simulink model "Bossi_Emanuele_EE460S3D_R99"  (R2025a)
settings: Solver=FixedStepDiscrete  StartTime=0.0  StopTime=120  FixedStep=dt0  RelTol=1e-3  EnableMultiTasking=on
PostLoadFcn:
  | %Set the size for the model
  | set_param(gcs,'Location',[10 10 1270 970])
  | %Set the zoom factor for the model
  | set_param(gcs,'ZoomFactor','100')
InitFcn:
  | tic
  | Bossi_Emanuele_EE460_Final
  | INIT_S3D_01
StartFcn:
  | tend0=toc;
  | tic;
StopFcn:
  | tend=toc;
  | disp(['Simulation time = ' num2str(tout(end)) ' sec'])
  | disp(['Real time = ' num2str(tend) ' sec'])
  | title('DONE')
  | SCORE=round((max(0,120-tout(end)-tend0))*4+10*(40-FuelBurned)+sum(100*double(PDONE)-100*double(PDONE<.5)));
  | PlotS3D(PlotInput);
  | text(15,22,['S: ' num2str(SCORE)]);
  | % Reset color scheme back to normal defaults
  | figure()
  | blkwhitebg('w');
  | close
values from neighbouring files (symbols this model uses):
  A_obs = [ 0  1  0  0  0  0 ... (first row only)    [Bossi_Emanuele_EE460_Final.m]
  B_obs = [ 0     0     0 ... (first row only)    [Bossi_Emanuele_EE460_Final.m]
  C_obs = [ 1 0 0 0 0 0 ... (first row only)    [Bossi_Emanuele_EE460_Final.m]
  d2r = pi/180    (= 0.0174532925199)    [INIT_S3D_01.m]
  D_obs = [ 0     0     0 ... (first row only)    [Bossi_Emanuele_EE460_Final.m]
  dt = 0.01    [INIT_S3D_01.m]
  dt0 = 0.001    [INIT_S3D_01.m]
  fr = 100    [INIT_S3D_01.m]
  G = [1,  1, -1, -1,  0,  0,  0,  0 ... (first row only)    [Bossi_Emanuele_EE460_Final.m]
  G_obs = eye(6)    [Bossi_Emanuele_EE460_Final.m]
  HM_S = 250    [INIT_S3D_01.m]
  HM_U = 500    [INIT_S3D_01.m]
  J = Jbase+JC0+JF+M*(Xcg^2+Ycg^2)    [INIT_S3D_01.m]
  Jbase = JC1+4*Ja+2*Ma*da^2+2*Ma*db^2    [INIT_S3D_01.m]
  JC0 = MC0/2    (= 10.2101761242)    [INIT_S3D_01.m]
  Kdtheta = 2 * zeta_th * wn_th * J_eff    [Bossi_Emanuele_EE460_Final.m]
  Kdtheta_fail = 2 * zeta_th_fail * wn_th_fail * J_eff    [Bossi_Emanuele_EE460_Final.m]
  Kdx = 2 * zeta_xy * wn_xy * M_eff    [Bossi_Emanuele_EE460_Final.m]
  Kdx_fail = 2 * zeta_xy_fail * wn_xy_fail * M_eff    [Bossi_Emanuele_EE460_Final.m]
  Kdy = 2 * zeta_xy * wn_xy * M_eff    [Bossi_Emanuele_EE460_Final.m]
  Kdy_fail = 2 * zeta_xy_fail * wn_xy_fail * M_eff    [Bossi_Emanuele_EE460_Final.m]
  Kptheta = J_eff * wn_th^2    [Bossi_Emanuele_EE460_Final.m]
  Kptheta_fail = J_eff * wn_th_fail^2    [Bossi_Emanuele_EE460_Final.m]
  Kpx = M_eff * wn_xy^2    [Bossi_Emanuele_EE460_Final.m]
  Kpx_fail = M_eff * wn_xy_fail^2    [Bossi_Emanuele_EE460_Final.m]
  Kpy = M_eff * wn_xy^2    [Bossi_Emanuele_EE460_Final.m]
  Kpy_fail = M_eff * wn_xy_fail^2    [Bossi_Emanuele_EE460_Final.m]
  L13 = sqrt(10)    [INIT_S3D_01.m]
  L24 = sqrt(6.25)    [INIT_S3D_01.m]
  LVL = LVL12    [INIT_S3D_01.m]
  M = MC+M1+M2+M3+M4+4*Ma    [INIT_S3D_01.m]
  M1 = LVL.M1    [INIT_S3D_01.m]
  M2 = LVL.M2    [INIT_S3D_01.m]
  M3 = LVL.M3    [INIT_S3D_01.m]
  M4 = LVL.M4    [INIT_S3D_01.m]
  max_qddot = [max_qddot_x; max_qddot_y; max_qddot_theta]    [Bossi_Emanuele_EE460_Final.m]
  mdti = (1/300)    (= 0.00333333333333)    [INIT_S3D_01.m]
  P = [1  1 -1 -1  0  0  0  0 ... (first row only)    [Bossi_Emanuele_EE460_Final.m]
  Pdata = [LVL.P1 LVL.P2 LVL.P3 LVL.P4]    [INIT_S3D_01.m]    (also in PlotS3D.m = R*[xt1;yt1+[0 3*tt*TV(idx-13)*TSIG(idx-13) 0]])
  PTvec = [Pdata(:,1);Pdata(:,2);Pdata(:,3);Pdata(:,4) ... (first row only)    [INIT_S3D_01.m]
  Q_obs = eye(6)    [Bossi_Emanuele_EE460_Final.m]
  r2d = 180/pi    (= 57.2957795131)    [INIT_S3D_01.m]
  r_bang = 0.5    [Bossi_Emanuele_EE460_Final.m]
  Sconfig = 1    [Bossi_Emanuele_EE460_Final.m]
  SLIM = [-100 100 ... (first row only)    [INIT_S3D_01.m]
  SQ = [.005 .01 .004 .005 .01 .004 .02 .01 .4]'    [INIT_S3D_01.m]
  SSF = 1./SQ    [INIT_S3D_01.m]
  tau = 0.5    [Bossi_Emanuele_EE460_Final.m]
  TOLdata = [LVL.P1tol LVL.P2tol LVL.P3tol LVL.P4tol]    [INIT_S3D_01.m]
  ULIM = [[Umin Umax];0 0;0 0]    [INIT_S3D_01.m]
undefined symbols (not defined in the file or in its folder): den_lp, den_lp2, DiscIntNeverNeededParam, dt1_bang_3, dt2_bang_3, dtc_bang_3, num_lp, num_lp2, q0_1
libraries: simulink x87, matrix_library x4, sl3dlib x1, aerolibutil x1, aerolibanimutils x1
(part 5 of 8)

== system Bossi_Emanuele_EE460S3D_R99/S3D_Plant/Sensors/CASE2/Ypos1 ==
  X : Inport
  Abs : Abs  SaturateOnIntegerOverflow=off
  Bus Selector3 : BusSelector  OutputSignals=y_m
  CURRENT : Subsystem  TreatAsAtomicUnit=on
  Compare To Constant : simulink/Logic and Bit Operations/Compare To Constant  relop=<=  const=0.5  OutDataTypeStr=boolean
  Constant1 : Constant  Value=LVL.Sfail(4)  SampleTime=dt0
  Constant2 : Constant  Value=LVL.Sft(4,1)+rand*(LVL.Sft(4,2)-LVL.Sft(4,1))  SampleTime=dt0
  Digital Clock : DigitalClock  SampleTime=dt0
  Gain : Gain  Gain=LVL.SN
  If : If  IfExpression=u1 < -0.5  ElseIfExpressions=u1 > 0.5 & u1 < 1.5
  Logical Operator : Logic  Operator=OR  AllPortsSameDT=off  OutDataTypeStr=boolean
  MAX : Subsystem  TreatAsAtomicUnit=on
  MIN : Subsystem  TreatAsAtomicUnit=on
  Merge : Merge  Inputs=3
  Quantizer : Quantizer  QuantizationInterval=SQ(4)  SampleTime=dt0
  Random Number : RandomNumber  Variance=LVL.SigSense(4)  Seed=4  SampleTime=dt0
  Relational Operator : RelationalOperator  Operator=<  OutDataTypeStr=boolean  InputSameDT=off
  Saturation : Saturate  UpperLimit=SLIM(4,2)  LowerLimit=SLIM(4,1)
  Sum : Sum  Inputs=|++
  Switch : Switch  Criteria=u2 > Threshold  SaturateOnIntegerOverflow=off  InputSameDT=off
  Unit Delay : UnitDelay  SampleTime=dt0  HasFrameUpgradeWarning=on
  y1 : Outport
  wires:
  Saturation/1 -> Quantizer/1
  Compare To Constant/1 -> Logical Operator/2
  Abs/1 -> Compare To Constant/1
  Constant1/1 -> If/1, Abs/1
  Logical Operator/1 -> Switch/2
  Relational Operator/1 -> Logical Operator/1
  Sum/1 -> Switch/1
  Bus Selector3/1 -> Sum/1  "<y_m>"
  Gain/1 -> Sum/2
  Random Number/1 -> Gain/1
  Merge/1 -> Switch/3
  MIN/1(Out1) -> Merge/1
  CURRENT/1(Out1) -> Merge/3
  X/1 -> Bus Selector3/1
  Constant2/1 -> Relational Operator/2
  MAX/1(Out1) -> Merge/2
  Unit Delay/1 -> CURRENT/1(In1)
  If/3 -> CURRENT/Action
  Digital Clock/1 -> Relational Operator/1
  Switch/1 -> Saturation/1
  If/2 -> MAX/Action
  If/1 -> MIN/Action
  Quantizer/1 -> Unit Delay/1, y1/1

== system Bossi_Emanuele_EE460S3D_R99/S3D_Plant/Sensors/CASE2/Ypos2 ==
  X : Inport
  Abs : Abs  SaturateOnIntegerOverflow=off
  Bus Selector3 : BusSelector  OutputSignals=y_m
  CURRENT : Subsystem  TreatAsAtomicUnit=on
  Compare To Constant : simulink/Logic and Bit Operations/Compare To Constant  relop=<=  const=0.5  OutDataTypeStr=boolean
  Constant1 : Constant  Value=LVL.Sfail(5)  SampleTime=dt0
  Constant2 : Constant  Value=LVL.Sft(5,1)+rand*(LVL.Sft(5,2)-LVL.Sft(5,1))  SampleTime=dt0
  Digital Clock : DigitalClock  SampleTime=dt0
  Gain : Gain  Gain=LVL.SN
  If : If  IfExpression=u1 < -0.5  ElseIfExpressions=u1 > 0.5 & u1 < 1.5
  Logical Operator : Logic  Operator=OR  AllPortsSameDT=off  OutDataTypeStr=boolean
  MAX : Subsystem  TreatAsAtomicUnit=on
  MIN : Subsystem  TreatAsAtomicUnit=on
  Merge : Merge  Inputs=3
  Quantizer : Quantizer  QuantizationInterval=SQ(4)  SampleTime=dt0
  Random Number : RandomNumber  Variance=LVL.SigSense(4)  Seed=5  SampleTime=dt0
  Relational Operator : RelationalOperator  Operator=<  OutDataTypeStr=boolean  InputSameDT=off
  Saturation : Saturate  UpperLimit=SLIM(4,2)  LowerLimit=SLIM(4,1)
  Sum : Sum  Inputs=|++
  Switch : Switch  Criteria=u2 > Threshold  SaturateOnIntegerOverflow=off  InputSameDT=off
  Unit Delay : UnitDelay  SampleTime=dt0  HasFrameUpgradeWarning=on
  y1 : Outport
  wires:
  Saturation/1 -> Quantizer/1
  Quantizer/1 -> y1/1, Unit Delay/1
  If/1 -> MIN/Action
  If/2 -> MAX/Action
  Switch/1 -> Saturation/1
  Digital Clock/1 -> Relational Operator/1
  If/3 -> CURRENT/Action
  Unit Delay/1 -> CURRENT/1(In1)
  MAX/1(Out1) -> Merge/2
  Constant2/1 -> Relational Operator/2
  X/1 -> Bus Selector3/1
  CURRENT/1(Out1) -> Merge/3
  MIN/1(Out1) -> Merge/1
  Merge/1 -> Switch/3
  Random Number/1 -> Gain/1
  Gain/1 -> Sum/2
  Bus Selector3/1 -> Sum/1  "<y_m>"
  Sum/1 -> Switch/1
  Relational Operator/1 -> Logical Operator/1
  Logical Operator/1 -> Switch/2
  Constant1/1 -> Abs/1, If/1
  Abs/1 -> Compare To Constant/1
  Compare To Constant/1 -> Logical Operator/2

== system Bossi_Emanuele_EE460S3D_R99/S3D_Plant/Sensors/CASE2/Yvel ==
  X : Inport
  Abs : Abs  SaturateOnIntegerOverflow=off
  Bus Selector3 : BusSelector  OutputSignals=ydt_mps
  CURRENT : Subsystem  TreatAsAtomicUnit=on
  Compare To Constant : simulink/Logic and Bit Operations/Compare To Constant  relop=<=  const=0.5  OutDataTypeStr=boolean
  Constant1 : Constant  Value=LVL.Sfail(6)  SampleTime=dt0
  Constant2 : Constant  Value=LVL.Sft(6,1)+rand*(LVL.Sft(6,2)-LVL.Sft(6,1))  SampleTime=dt0
  Digital Clock : DigitalClock  SampleTime=dt0
  Gain : Gain  Gain=LVL.SN
  If : If  IfExpression=u1 < -0.5  ElseIfExpressions=u1 > 0.5 & u1 < 1.5
  Logical Operator : Logic  Operator=OR  AllPortsSameDT=off  OutDataTypeStr=boolean
  MAX : Subsystem  TreatAsAtomicUnit=on
  MIN : Subsystem  TreatAsAtomicUnit=on
  Merge : Merge  Inputs=3
  Quantizer : Quantizer  QuantizationInterval=SQ(5)  SampleTime=dt0
  Random Number : RandomNumber  Variance=LVL.SigSense(5)  Seed=6  SampleTime=dt0
  Relational Operator : RelationalOperator  Operator=<  OutDataTypeStr=boolean  InputSameDT=off
  Saturation : Saturate  UpperLimit=SLIM(5,2)  LowerLimit=SLIM(5,1)
  Sum : Sum  Inputs=|++
  Switch : Switch  Criteria=u2 > Threshold  SaturateOnIntegerOverflow=off  InputSameDT=off
  Unit Delay : UnitDelay  SampleTime=dt0  HasFrameUpgradeWarning=on
  ydt1 : Outport
  wires:
  Saturation/1 -> Quantizer/1
  If/1 -> MIN/Action
  If/2 -> MAX/Action
  Switch/1 -> Saturation/1
  Digital Clock/1 -> Relational Operator/1
  If/3 -> CURRENT/Action
  Unit Delay/1 -> CURRENT/1(In1)
  MAX/1(Out1) -> Merge/2
  Constant2/1 -> Relational Operator/2
  X/1 -> Bus Selector3/1
  CURRENT/1(Out1) -> Merge/3
  MIN/1(Out1) -> Merge/1
  Merge/1 -> Switch/3
  Random Number/1 -> Gain/1
  Gain/1 -> Sum/2
  Bus Selector3/1 -> Sum/1  "<ydt_mps>"
  Sum/1 -> Switch/1
  Relational Operator/1 -> Logical Operator/1
  Logical Operator/1 -> Switch/2
  Constant1/1 -> Abs/1, If/1
  Abs/1 -> Compare To Constant/1
  Compare To Constant/1 -> Logical Operator/2
  Quantizer/1 -> ydt1/1, Unit Delay/1

== system Bossi_Emanuele_EE460S3D_R99/S3D_Plant/Sensors/CASE3/THTpos1 ==
  X : Inport
  Abs : Abs  SaturateOnIntegerOverflow=off
  Bus Selector3 : BusSelector  OutputSignals=tht_rad
  CURRENT : Subsystem  TreatAsAtomicUnit=on
  Compare To Constant : simulink/Logic and Bit Operations/Compare To Constant  relop=<=  const=0.5  OutDataTypeStr=boolean
  Constant1 : Constant  Value=LVL.Sfail(7)  SampleTime=dt0
  Constant2 : Constant  Value=LVL.Sft(7,1)+rand*(LVL.Sft(7,2)-LVL.Sft(7,1))  SampleTime=dt0
  Digital Clock : DigitalClock  SampleTime=dt0
  Gain : Gain  Gain=LVL.SN
  Gain4 : Gain  Gain=r2d
  If : If  IfExpression=u1 < -0.5  ElseIfExpressions=u1 > 0.5 & u1 < 1.5
  Logical Operator : Logic  Operator=OR  AllPortsSameDT=off  OutDataTypeStr=boolean
  MAX : Subsystem  TreatAsAtomicUnit=on
  MIN : Subsystem  TreatAsAtomicUnit=on
  Merge : Merge  Inputs=3
  Quantizer : Quantizer  QuantizationInterval=SQ(7)  SampleTime=dt0
  Random Number : RandomNumber  Variance=LVL.SigSense(7)  Seed=7  SampleTime=dt0
  Relational Operator : RelationalOperator  Operator=<  OutDataTypeStr=boolean  InputSameDT=off
  Saturation : Saturate  UpperLimit=SLIM(7,2)  LowerLimit=SLIM(7,1)
  Sum : Sum  Inputs=|++
  Switch : Switch  Criteria=u2 > Threshold  SaturateOnIntegerOverflow=off  InputSameDT=off
  Unit Delay : UnitDelay  SampleTime=dt0  HasFrameUpgradeWarning=on
  tht1 : Outport
  wires:
  Saturation/1 -> Quantizer/1
  Switch/1 -> Saturation/1
  Quantizer/1 -> Unit Delay/1, tht1/1
  Gain4/1 -> Sum/1
  Compare To Constant/1 -> Logical Operator/2
  Abs/1 -> Compare To Constant/1
  Constant1/1 -> If/1, Abs/1
  Logical Operator/1 -> Switch/2
  Relational Operator/1 -> Logical Operator/1
  Sum/1 -> Switch/1
  Bus Selector3/1 -> Gain4/1  "<tht_rad>"
  Gain/1 -> Sum/2
  Random Number/1 -> Gain/1
  Merge/1 -> Switch/3
  MIN/1(Out1) -> Merge/1
  CURRENT/1(Out1) -> Merge/3
  X/1 -> Bus Selector3/1
  Constant2/1 -> Relational Operator/2
  MAX/1(Out1) -> Merge/2
  Unit Delay/1 -> CURRENT/1(In1)
  If/3 -> CURRENT/Action
  Digital Clock/1 -> Relational Operator/1
  If/2 -> MAX/Action
  If/1 -> MIN/Action

== system Bossi_Emanuele_EE460S3D_R99/S3D_Plant/Sensors/CASE3/THTpos2 ==
  X : Inport
  Abs : Abs  SaturateOnIntegerOverflow=off
  Bus Selector3 : BusSelector  OutputSignals=tht_rad
  CURRENT : Subsystem  TreatAsAtomicUnit=on
  Compare To Constant : simulink/Logic and Bit Operations/Compare To Constant  relop=<=  const=0.5  OutDataTypeStr=boolean
  Constant1 : Constant  Value=LVL.Sfail(8)  SampleTime=dt0
  Constant2 : Constant  Value=LVL.Sft(8,1)+rand*(LVL.Sft(8,2)-LVL.Sft(8,1))  SampleTime=dt0
  Digital Clock : DigitalClock  SampleTime=dt0
  Gain : Gain  Gain=LVL.SN
  Gain4 : Gain  Gain=r2d
  If : If  IfExpression=u1 < -0.5  ElseIfExpressions=u1 > 0.5 & u1 < 1.5
  Logical Operator : Logic  Operator=OR  AllPortsSameDT=off  OutDataTypeStr=boolean
  MAX : Subsystem  TreatAsAtomicUnit=on
  MIN : Subsystem  TreatAsAtomicUnit=on
  Merge : Merge  Inputs=3
  Quantizer : Quantizer  QuantizationInterval=SQ(7)  SampleTime=dt0
  Random Number : RandomNumber  Variance=LVL.SigSense(7)  Seed=8  SampleTime=dt0
  Relational Operator : RelationalOperator  Operator=<  OutDataTypeStr=boolean  InputSameDT=off
  Saturation : Saturate  UpperLimit=SLIM(7,2)  LowerLimit=SLIM(7,1)
  Sum : Sum  Inputs=|++
  Switch : Switch  Criteria=u2 > Threshold  SaturateOnIntegerOverflow=off  InputSameDT=off
  Unit Delay : UnitDelay  SampleTime=dt0  HasFrameUpgradeWarning=on
  tht1 : Outport
  wires:
  Saturation/1 -> Quantizer/1
  If/1 -> MIN/Action
  If/2 -> MAX/Action
  Digital Clock/1 -> Relational Operator/1
  If/3 -> CURRENT/Action
  Unit Delay/1 -> CURRENT/1(In1)
  MAX/1(Out1) -> Merge/2
  Constant2/1 -> Relational Operator/2
  X/1 -> Bus Selector3/1
  CURRENT/1(Out1) -> Merge/3
  MIN/1(Out1) -> Merge/1
  Merge/1 -> Switch/3
  Random Number/1 -> Gain/1
  Gain/1 -> Sum/2
  Bus Selector3/1 -> Gain4/1  "<tht_rad>"
  Sum/1 -> Switch/1
  Relational Operator/1 -> Logical Operator/1
  Logical Operator/1 -> Switch/2
  Constant1/1 -> Abs/1, If/1
  Abs/1 -> Compare To Constant/1
  Compare To Constant/1 -> Logical Operator/2
  Gain4/1 -> Sum/1
  Switch/1 -> Saturation/1
  Quantizer/1 -> Unit Delay/1, tht1/1

== system Bossi_Emanuele_EE460S3D_R99/S3D_Plant/Sensors/CASE3/THTpos3 ==
  X : Inport
  Abs : Abs  SaturateOnIntegerOverflow=off
  Bus Selector3 : BusSelector  OutputSignals=tht_rad
  CURRENT : Subsystem  TreatAsAtomicUnit=on
  Compare To Constant : simulink/Logic and Bit Operations/Compare To Constant  relop=<=  const=0.5  OutDataTypeStr=boolean
  Constant1 : Constant  Value=LVL.Sfail(9)  SampleTime=dt0
  Constant2 : Constant  Value=LVL.Sft(9,1)+rand*(LVL.Sft(9,2)-LVL.Sft(9,1))  SampleTime=dt0
  Digital Clock : DigitalClock  SampleTime=dt0
  Gain : Gain  Gain=LVL.SN
  Gain4 : Gain  Gain=r2d
  If : If  IfExpression=u1 < -0.5  ElseIfExpressions=u1 > 0.5 & u1 < 1.5
  Logical Operator : Logic  Operator=OR  AllPortsSameDT=off  OutDataTypeStr=boolean
  MAX : Subsystem  TreatAsAtomicUnit=on
  MIN : Subsystem  TreatAsAtomicUnit=on
  Merge : Merge  Inputs=3
  Quantizer : Quantizer  QuantizationInterval=SQ(7)  SampleTime=dt0
  Random Number : RandomNumber  Variance=LVL.SigSense(7)  Seed=9  SampleTime=dt0
  Relational Operator : RelationalOperator  Operator=<  OutDataTypeStr=boolean  InputSameDT=off
  Saturation : Saturate  UpperLimit=SLIM(7,2)  LowerLimit=SLIM(7,1)
  Sum : Sum  Inputs=|++
  Switch : Switch  Criteria=u2 > Threshold  SaturateOnIntegerOverflow=off  InputSameDT=off
  Unit Delay : UnitDelay  SampleTime=dt0  HasFrameUpgradeWarning=on
  tht1 : Outport
  wires:
  Saturation/1 -> Quantizer/1
  Switch/1 -> Saturation/1
  Quantizer/1 -> Unit Delay/1, tht1/1
  Gain4/1 -> Sum/1
  Compare To Constant/1 -> Logical Operator/2
  Abs/1 -> Compare To Constant/1
  Constant1/1 -> If/1, Abs/1
  Logical Operator/1 -> Switch/2
  Relational Operator/1 -> Logical Operator/1
  Sum/1 -> Switch/1
  Bus Selector3/1 -> Gain4/1  "<tht_rad>"
  Gain/1 -> Sum/2
  Random Number/1 -> Gain/1
  Merge/1 -> Switch/3
  MIN/1(Out1) -> Merge/1
  CURRENT/1(Out1) -> Merge/3
  X/1 -> Bus Selector3/1
  Constant2/1 -> Relational Operator/2
  MAX/1(Out1) -> Merge/2
  Unit Delay/1 -> CURRENT/1(In1)
  If/3 -> CURRENT/Action
  Digital Clock/1 -> Relational Operator/1
  If/2 -> MAX/Action
  If/1 -> MIN/Action

== system Bossi_Emanuele_EE460S3D_R99/S3D_Plant/Sensors/CASE3/Xpos1 ==
  X : Inport
  Abs : Abs  SaturateOnIntegerOverflow=off
  Bus Selector3 : BusSelector  OutputSignals=x_m
  CURRENT : Subsystem  TreatAsAtomicUnit=on
  Compare To Constant : simulink/Logic and Bit Operations/Compare To Constant  relop=<=  const=0.5  OutDataTypeStr=boolean
  Constant1 : Constant  Value=LVL.Sfail(1)  SampleTime=dt0
  Constant2 : Constant  Value=LVL.Sft(1,1)+rand*(LVL.Sft(1,2)-LVL.Sft(1,1))  SampleTime=dt0
  Digital Clock : DigitalClock  SampleTime=dt0
  Gain : Gain  Gain=LVL.SN
  If : If  IfExpression=u1 < -0.5  ElseIfExpressions=u1 > 0.5 & u1 < 1.5
  Logical Operator : Logic  Operator=OR  AllPortsSameDT=off  OutDataTypeStr=boolean
  MAX : Subsystem  TreatAsAtomicUnit=on
  MIN : Subsystem  TreatAsAtomicUnit=on
  Merge : Merge  Inputs=3
  Quantizer : Quantizer  QuantizationInterval=SQ(1)  SampleTime=dt0
  Random Number : RandomNumber  Variance=LVL.SigSense(1)  Seed=1  SampleTime=dt0
  Relational Operator : RelationalOperator  Operator=<  OutDataTypeStr=boolean  InputSameDT=off
  Saturation : Saturate  UpperLimit=SLIM(1,2)  LowerLimit=SLIM(1,1)
  Sum : Sum  Inputs=|++
  Switch : Switch  Criteria=u2 > Threshold  SaturateOnIntegerOverflow=off  InputSameDT=off
  Unit Delay : UnitDelay  SampleTime=dt0  HasFrameUpgradeWarning=on
  x1 : Outport
  wires:
  Saturation/1 -> Quantizer/1
  Quantizer/1 -> Unit Delay/1, x1/1
  Compare To Constant/1 -> Logical Operator/2
  Abs/1 -> Compare To Constant/1
  Constant1/1 -> If/1, Abs/1
  Logical Operator/1 -> Switch/2
  Relational Operator/1 -> Logical Operator/1
  Sum/1 -> Switch/1
  Bus Selector3/1 -> Sum/1  "<x_m>"
  Gain/1 -> Sum/2
  Random Number/1 -> Gain/1
  Merge/1 -> Switch/3
  MIN/1(Out1) -> Merge/1
  CURRENT/1(Out1) -> Merge/3
  X/1 -> Bus Selector3/1
  Constant2/1 -> Relational Operator/2
  MAX/1(Out1) -> Merge/2
  Unit Delay/1 -> CURRENT/1(In1)
  If/3 -> CURRENT/Action
  Digital Clock/1 -> Relational Operator/1
  Switch/1 -> Saturation/1
  If/2 -> MAX/Action
  If/1 -> MIN/Action

== system Bossi_Emanuele_EE460S3D_R99/S3D_Plant/Sensors/CASE3/Xpos2 ==
  X : Inport
  Abs : Abs  SaturateOnIntegerOverflow=off
  Bus Selector3 : BusSelector  OutputSignals=x_m
  CURRENT : Subsystem  TreatAsAtomicUnit=on
  Compare To Constant : simulink/Logic and Bit Operations/Compare To Constant  relop=<=  const=0.5  OutDataTypeStr=boolean
  Constant1 : Constant  Value=LVL.Sfail(2)  SampleTime=dt0
  Constant2 : Constant  Value=LVL.Sft(2,1)+rand*(LVL.Sft(2,2)-LVL.Sft(2,1))  SampleTime=dt0
  Digital Clock : DigitalClock  SampleTime=dt0
  Gain : Gain  Gain=LVL.SN
  If : If  IfExpression=u1 < -0.5  ElseIfExpressions=u1 > 0.5 & u1 < 1.5
  Logical Operator : Logic  Operator=OR  AllPortsSameDT=off  OutDataTypeStr=boolean
  MAX : Subsystem  TreatAsAtomicUnit=on
  MIN : Subsystem  TreatAsAtomicUnit=on
  Merge : Merge  Inputs=3
  Quantizer : Quantizer  QuantizationInterval=SQ(1)  SampleTime=dt0
  Random Number : RandomNumber  Variance=LVL.SigSense(1)  Seed=2  SampleTime=dt0
  Relational Operator : RelationalOperator  Operator=<  OutDataTypeStr=boolean  InputSameDT=off
  Saturation : Saturate  UpperLimit=SLIM(1,2)  LowerLimit=SLIM(1,1)
  Sum : Sum  Inputs=|++
  Switch : Switch  Criteria=u2 > Threshold  SaturateOnIntegerOverflow=off  InputSameDT=off
  Unit Delay : UnitDelay  SampleTime=dt0  HasFrameUpgradeWarning=on
  xdt1 : Outport
  wires:
  Saturation/1 -> Quantizer/1
  Quantizer/1 -> xdt1/1, Unit Delay/1
  If/1 -> MIN/Action
  If/2 -> MAX/Action
  Switch/1 -> Saturation/1
  Digital Clock/1 -> Relational Operator/1
  If/3 -> CURRENT/Action
  Unit Delay/1 -> CURRENT/1(In1)
  MAX/1(Out1) -> Merge/2
  Constant2/1 -> Relational Operator/2
  X/1 -> Bus Selector3/1
  CURRENT/1(Out1) -> Merge/3
  MIN/1(Out1) -> Merge/1
  Merge/1 -> Switch/3
  Random Number/1 -> Gain/1
  Gain/1 -> Sum/2
  Bus Selector3/1 -> Sum/1  "<x_m>"
  Sum/1 -> Switch/1
  Relational Operator/1 -> Logical Operator/1
  Logical Operator/1 -> Switch/2
  Constant1/1 -> Abs/1, If/1
  Abs/1 -> Compare To Constant/1
  Compare To Constant/1 -> Logical Operator/2

== system Bossi_Emanuele_EE460S3D_R99/S3D_Plant/Sensors/CASE3/Xpos3 ==
  X : Inport
  Abs : Abs  SaturateOnIntegerOverflow=off
  Bus Selector3 : BusSelector  OutputSignals=x_m
  CURRENT : Subsystem  TreatAsAtomicUnit=on
  Compare To Constant : simulink/Logic and Bit Operations/Compare To Constant  relop=<=  const=0.5  OutDataTypeStr=boolean
  Constant1 : Constant  Value=LVL.Sfail(3)  SampleTime=dt0
  Constant2 : Constant  Value=LVL.Sft(3,1)+rand*(LVL.Sft(3,2)-LVL.Sft(3,1))  SampleTime=dt0
  Digital Clock : DigitalClock  SampleTime=dt0
  Gain : Gain  Gain=LVL.SN
  If : If  IfExpression=u1 < -0.5  ElseIfExpressions=u1 > 0.5 & u1 < 1.5
  Logical Operator : Logic  Operator=OR  AllPortsSameDT=off  OutDataTypeStr=boolean
  MAX : Subsystem  TreatAsAtomicUnit=on
  MIN : Subsystem  TreatAsAtomicUnit=on
  Merge : Merge  Inputs=3
  Quantizer : Quantizer  QuantizationInterval=SQ(1)  SampleTime=dt0
  Random Number : RandomNumber  Variance=LVL.SigSense(1)  Seed=3  SampleTime=dt0
  Relational Operator : RelationalOperator  Operator=<  OutDataTypeStr=boolean  InputSameDT=off
  Saturation : Saturate  UpperLimit=SLIM(1,2)  LowerLimit=SLIM(1,1)
  Sum : Sum  Inputs=|++
  Switch : Switch  Criteria=u2 > Threshold  SaturateOnIntegerOverflow=off  InputSameDT=off
  Unit Delay : UnitDelay  SampleTime=dt0  HasFrameUpgradeWarning=on
  xddt1 : Outport
  wires:
  Saturation/1 -> Quantizer/1
  Quantizer/1 -> Unit Delay/1, xddt1/1
  Compare To Constant/1 -> Logical Operator/2
  Abs/1 -> Compare To Constant/1
  Constant1/1 -> If/1, Abs/1
  Logical Operator/1 -> Switch/2
  Relational Operator/1 -> Logical Operator/1
  Sum/1 -> Switch/1
  Bus Selector3/1 -> Sum/1  "<x_m>"
  Gain/1 -> Sum/2
  Random Number/1 -> Gain/1
  Merge/1 -> Switch/3
  MIN/1(Out1) -> Merge/1
  CURRENT/1(Out1) -> Merge/3
  X/1 -> Bus Selector3/1
  Constant2/1 -> Relational Operator/2
  MAX/1(Out1) -> Merge/2
  Unit Delay/1 -> CURRENT/1(In1)
  If/3 -> CURRENT/Action
  Digital Clock/1 -> Relational Operator/1
  Switch/1 -> Saturation/1
  If/2 -> MAX/Action
  If/1 -> MIN/Action

== system Bossi_Emanuele_EE460S3D_R99/S3D_Plant/Sensors/CASE3/Ypos1 ==
  X : Inport
  Abs : Abs  SaturateOnIntegerOverflow=off
  Bus Selector3 : BusSelector  OutputSignals=y_m
  CURRENT : Subsystem  TreatAsAtomicUnit=on
  Compare To Constant : simulink/Logic and Bit Operations/Compare To Constant  relop=<=  const=0.5  OutDataTypeStr=boolean
  Constant1 : Constant  Value=LVL.Sfail(4)  SampleTime=dt0
  Constant2 : Constant  Value=LVL.Sft(4,1)+rand*(LVL.Sft(4,2)-LVL.Sft(4,1))  SampleTime=dt0
  Digital Clock : DigitalClock  SampleTime=dt0
  Gain : Gain  Gain=LVL.SN
  If : If  IfExpression=u1 < -0.5  ElseIfExpressions=u1 > 0.5 & u1 < 1.5
  Logical Operator : Logic  Operator=OR  AllPortsSameDT=off  OutDataTypeStr=boolean
  MAX : Subsystem  TreatAsAtomicUnit=on
  MIN : Subsystem  TreatAsAtomicUnit=on
  Merge : Merge  Inputs=3
  Quantizer : Quantizer  QuantizationInterval=SQ(4)  SampleTime=dt0
  Random Number : RandomNumber  Variance=LVL.SigSense(4)  Seed=4  SampleTime=dt0
  Relational Operator : RelationalOperator  Operator=<  OutDataTypeStr=boolean  InputSameDT=off
  Saturation : Saturate  UpperLimit=SLIM(4,2)  LowerLimit=SLIM(4,1)
  Sum : Sum  Inputs=|++
  Switch : Switch  Criteria=u2 > Threshold  SaturateOnIntegerOverflow=off  InputSameDT=off
  Unit Delay : UnitDelay  SampleTime=dt0  HasFrameUpgradeWarning=on
  y1 : Outport
  wires:
  Saturation/1 -> Quantizer/1
  Quantizer/1 -> y1/1, Unit Delay/1
  If/1 -> MIN/Action
  If/2 -> MAX/Action
  Switch/1 -> Saturation/1
  Digital Clock/1 -> Relational Operator/1
  If/3 -> CURRENT/Action
  Unit Delay/1 -> CURRENT/1(In1)
  MAX/1(Out1) -> Merge/2
  Constant2/1 -> Relational Operator/2
  X/1 -> Bus Selector3/1
  CURRENT/1(Out1) -> Merge/3
  MIN/1(Out1) -> Merge/1
  Merge/1 -> Switch/3
  Random Number/1 -> Gain/1
  Gain/1 -> Sum/2
  Bus Selector3/1 -> Sum/1  "<y_m>"
  Sum/1 -> Switch/1
  Relational Operator/1 -> Logical Operator/1
  Logical Operator/1 -> Switch/2
  Constant1/1 -> Abs/1, If/1
  Abs/1 -> Compare To Constant/1
  Compare To Constant/1 -> Logical Operator/2

== system Bossi_Emanuele_EE460S3D_R99/S3D_Plant/Sensors/CASE3/Ypos2 ==
  X : Inport
  Abs : Abs  SaturateOnIntegerOverflow=off
  Bus Selector3 : BusSelector  OutputSignals=y_m
  CURRENT : Subsystem  TreatAsAtomicUnit=on
  Compare To Constant : simulink/Logic and Bit Operations/Compare To Constant  relop=<=  const=0.5  OutDataTypeStr=boolean
  Constant1 : Constant  Value=LVL.Sfail(5)  SampleTime=dt0
  Constant2 : Constant  Value=LVL.Sft(5,1)+rand*(LVL.Sft(5,2)-LVL.Sft(5,1))  SampleTime=dt0
  Digital Clock : DigitalClock  SampleTime=dt0
  Gain : Gain  Gain=LVL.SN
  If : If  IfExpression=u1 < -0.5  ElseIfExpressions=u1 > 0.5 & u1 < 1.5
  Logical Operator : Logic  Operator=OR  AllPortsSameDT=off  OutDataTypeStr=boolean
  MAX : Subsystem  TreatAsAtomicUnit=on
  MIN : Subsystem  TreatAsAtomicUnit=on
  Merge : Merge  Inputs=3
  Quantizer : Quantizer  QuantizationInterval=SQ(4)  SampleTime=dt0
  Random Number : RandomNumber  Variance=LVL.SigSense(4)  Seed=5  SampleTime=dt0
  Relational Operator : RelationalOperator  Operator=<  OutDataTypeStr=boolean  InputSameDT=off
  Saturation : Saturate  UpperLimit=SLIM(4,2)  LowerLimit=SLIM(4,1)
  Sum : Sum  Inputs=|++
  Switch : Switch  Criteria=u2 > Threshold  SaturateOnIntegerOverflow=off  InputSameDT=off
  Unit Delay : UnitDelay  SampleTime=dt0  HasFrameUpgradeWarning=on
  y1 : Outport
  wires:
  Saturation/1 -> Quantizer/1
  Compare To Constant/1 -> Logical Operator/2
  Abs/1 -> Compare To Constant/1
  Constant1/1 -> If/1, Abs/1
  Logical Operator/1 -> Switch/2
  Relational Operator/1 -> Logical Operator/1
  Sum/1 -> Switch/1
  Bus Selector3/1 -> Sum/1  "<y_m>"
  Gain/1 -> Sum/2
  Random Number/1 -> Gain/1
  Merge/1 -> Switch/3
  MIN/1(Out1) -> Merge/1
  CURRENT/1(Out1) -> Merge/3
  X/1 -> Bus Selector3/1
  Constant2/1 -> Relational Operator/2
  MAX/1(Out1) -> Merge/2
  Unit Delay/1 -> CURRENT/1(In1)
  If/3 -> CURRENT/Action
  Digital Clock/1 -> Relational Operator/1
  Switch/1 -> Saturation/1
  If/2 -> MAX/Action
  If/1 -> MIN/Action
  Quantizer/1 -> Unit Delay/1, y1/1

== system Bossi_Emanuele_EE460S3D_R99/S3D_Plant/Sensors/CASE3/Ypos3 ==
  X : Inport
  Abs : Abs  SaturateOnIntegerOverflow=off
  Bus Selector3 : BusSelector  OutputSignals=y_m
  CURRENT : Subsystem  TreatAsAtomicUnit=on
  Compare To Constant : simulink/Logic and Bit Operations/Compare To Constant  relop=<=  const=0.5  OutDataTypeStr=boolean
  Constant1 : Constant  Value=LVL.Sfail(6)  SampleTime=dt0
  Constant2 : Constant  Value=LVL.Sft(6,1)+rand*(LVL.Sft(6,2)-LVL.Sft(6,1))  SampleTime=dt0
  Digital Clock : DigitalClock  SampleTime=dt0
  Gain : Gain  Gain=LVL.SN
  If : If  IfExpression=u1 < -0.5  ElseIfExpressions=u1 > 0.5 & u1 < 1.5
  Logical Operator : Logic  Operator=OR  AllPortsSameDT=off  OutDataTypeStr=boolean
  MAX : Subsystem  TreatAsAtomicUnit=on
  MIN : Subsystem  TreatAsAtomicUnit=on
  Merge : Merge  Inputs=3
  Quantizer : Quantizer  QuantizationInterval=SQ(4)  SampleTime=dt0
  Random Number : RandomNumber  Variance=LVL.SigSense(4)  Seed=6  SampleTime=dt0
  Relational Operator : RelationalOperator  Operator=<  OutDataTypeStr=boolean  InputSameDT=off
  Saturation : Saturate  UpperLimit=SLIM(4,2)  LowerLimit=SLIM(4,1)
  Sum : Sum  Inputs=|++
  Switch : Switch  Criteria=u2 > Threshold  SaturateOnIntegerOverflow=off  InputSameDT=off
  Unit Delay : UnitDelay  SampleTime=dt0  HasFrameUpgradeWarning=on
  y1 : Outport
  wires:
  Saturation/1 -> Quantizer/1
  Quantizer/1 -> y1/1, Unit Delay/1
  If/1 -> MIN/Action
  If/2 -> MAX/Action
  Switch/1 -> Saturation/1
  Digital Clock/1 -> Relational Operator/1
  If/3 -> CURRENT/Action
  Unit Delay/1 -> CURRENT/1(In1)
  MAX/1(Out1) -> Merge/2
  Constant2/1 -> Relational Operator/2
  X/1 -> Bus Selector3/1
  CURRENT/1(Out1) -> Merge/3
  MIN/1(Out1) -> Merge/1
  Merge/1 -> Switch/3
  Random Number/1 -> Gain/1
  Gain/1 -> Sum/2
  Bus Selector3/1 -> Sum/1  "<y_m>"
  Sum/1 -> Switch/1
  Relational Operator/1 -> Logical Operator/1
  Logical Operator/1 -> Switch/2
  Constant1/1 -> Abs/1, If/1
  Abs/1 -> Compare To Constant/1
  Compare To Constant/1 -> Logical Operator/2

== system Bossi_Emanuele_EE460S3D_R99/S3D_Plant/Sensors/HealthMonitoring/Subsystem ==
  In1 : Inport
  Compare To Constant : simulink/Logic and Bit Operations/Compare To Constant  relop=>=  const=HM_S  OutDataTypeStr=boolean
  Constant : Constant  Value=0
  Constant1 : Constant
  Logical Operator : Logic  Operator=OR  AllPortsSameDT=off  OutDataTypeStr=boolean
  Sum : Sum  Inputs=|+-  OutDataTypeStr=int32
  Sum1 : Sum  Inputs=|++
  Switch : Switch  Criteria=u2 > Threshold  Threshold=eps  SaturateOnIntegerOverflow=off  InputSameDT=off
  Unit Delay : UnitDelay  SampleTime=dt0  HasFrameUpgradeWarning=on
  Unit Delay1 : UnitDelay  SampleTime=dt0  HasFrameUpgradeWarning=on
  Unit Delay2 : UnitDelay  SampleTime=dt0  HasFrameUpgradeWarning=on
  Out1 : Outport
  wires:
  Logical Operator/1 -> Unit Delay2/1, Out1/1
  Constant1/1 -> Sum1/1
  Compare To Constant/1 -> Logical Operator/1
  Switch/1 -> Unit Delay1/1, Compare To Constant/1
  In1/1 -> Sum/1, Unit Delay/1
  Unit Delay2/1 -> Logical Operator/2
  Unit Delay/1 -> Sum/2
  Sum/1 -> Switch/2
  Sum1/1 -> Switch/3
  Unit Delay1/1 -> Sum1/2
  Constant/1 -> Switch/1

== system Bossi_Emanuele_EE460S3D_R99/S3D_Plant/Sensors/HealthMonitoring/Subsystem1 ==
  In1 : Inport
  Compare To Constant : simulink/Logic and Bit Operations/Compare To Constant  relop=>=  const=HM_S  OutDataTypeStr=boolean
  Constant : Constant  Value=0
  Constant1 : Constant
  Logical Operator : Logic  Operator=OR  AllPortsSameDT=off  OutDataTypeStr=boolean
  Sum : Sum  Inputs=|+-  OutDataTypeStr=int32
  Sum1 : Sum  Inputs=|++
  Switch : Switch  Criteria=u2 > Threshold  Threshold=eps  SaturateOnIntegerOverflow=off  InputSameDT=off
  Unit Delay : UnitDelay  SampleTime=dt0  HasFrameUpgradeWarning=on
  Unit Delay1 : UnitDelay  SampleTime=dt0  HasFrameUpgradeWarning=on
  Unit Delay2 : UnitDelay  SampleTime=dt0  HasFrameUpgradeWarning=on
  Out1 : Outport
  wires:
  Constant/1 -> Switch/1
  Unit Delay1/1 -> Sum1/2
  Sum1/1 -> Switch/3
  Sum/1 -> Switch/2
  Unit Delay/1 -> Sum/2
  Unit Delay2/1 -> Logical Operator/2
  In1/1 -> Unit Delay/1, Sum/1
  Switch/1 -> Compare To Constant/1, Unit Delay1/1
  Compare To Constant/1 -> Logical Operator/1
  Constant1/1 -> Sum1/1
  Logical Operator/1 -> Out1/1, Unit Delay2/1

== system Bossi_Emanuele_EE460S3D_R99/S3D_Plant/Sensors/HealthMonitoring/Subsystem2 ==
  In1 : Inport
  Compare To Constant : simulink/Logic and Bit Operations/Compare To Constant  relop=>=  const=HM_S  OutDataTypeStr=boolean
  Constant : Constant  Value=0
  Constant1 : Constant
  Logical Operator : Logic  Operator=OR  AllPortsSameDT=off  OutDataTypeStr=boolean
  Sum : Sum  Inputs=|+-  OutDataTypeStr=int32
  Sum1 : Sum  Inputs=|++
  Switch : Switch  Criteria=u2 > Threshold  Threshold=eps  SaturateOnIntegerOverflow=off  InputSameDT=off
  Unit Delay : UnitDelay  SampleTime=dt0  HasFrameUpgradeWarning=on
  Unit Delay1 : UnitDelay  SampleTime=dt0  HasFrameUpgradeWarning=on
  Unit Delay2 : UnitDelay  SampleTime=dt0  HasFrameUpgradeWarning=on
  Out1 : Outport
  wires:
  Logical Operator/1 -> Unit Delay2/1, Out1/1
  Constant1/1 -> Sum1/1
  Compare To Constant/1 -> Logical Operator/1
  Switch/1 -> Unit Delay1/1, Compare To Constant/1
  In1/1 -> Sum/1, Unit Delay/1
  Unit Delay2/1 -> Logical Operator/2
  Unit Delay/1 -> Sum/2
  Sum/1 -> Switch/2
  Sum1/1 -> Switch/3
  Unit Delay1/1 -> Sum1/2
  Constant/1 -> Switch/1

== system Bossi_Emanuele_EE460S3D_R99/S3D_Plant/Sensors/HealthMonitoring/Subsystem3 ==
  In1 : Inport
  Compare To Constant : simulink/Logic and Bit Operations/Compare To Constant  relop=>=  const=HM_S  OutDataTypeStr=boolean
  Constant : Constant  Value=0
  Constant1 : Constant
  Logical Operator : Logic  Operator=OR  AllPortsSameDT=off  OutDataTypeStr=boolean
  Sum : Sum  Inputs=|+-  OutDataTypeStr=int32
  Sum1 : Sum  Inputs=|++
  Switch : Switch  Criteria=u2 > Threshold  Threshold=eps  SaturateOnIntegerOverflow=off  InputSameDT=off
  Unit Delay : UnitDelay  SampleTime=dt0  HasFrameUpgradeWarning=on
  Unit Delay1 : UnitDelay  SampleTime=dt0  HasFrameUpgradeWarning=on
  Unit Delay2 : UnitDelay  SampleTime=dt0  HasFrameUpgradeWarning=on
  Out1 : Outport
  wires:
  Constant/1 -> Switch/1
  Unit Delay1/1 -> Sum1/2
  Sum1/1 -> Switch/3
  Sum/1 -> Switch/2
  Unit Delay/1 -> Sum/2
  Unit Delay2/1 -> Logical Operator/2
  In1/1 -> Unit Delay/1, Sum/1
  Switch/1 -> Compare To Constant/1, Unit Delay1/1
  Compare To Constant/1 -> Logical Operator/1
  Constant1/1 -> Sum1/1
  Logical Operator/1 -> Out1/1, Unit Delay2/1

== system Bossi_Emanuele_EE460S3D_R99/S3D_Plant/Sensors/HealthMonitoring/Subsystem4 ==
  In1 : Inport
  Compare To Constant : simulink/Logic and Bit Operations/Compare To Constant  relop=>=  const=HM_S  OutDataTypeStr=boolean
  Constant : Constant  Value=0
  Constant1 : Constant
  Logical Operator : Logic  Operator=OR  AllPortsSameDT=off  OutDataTypeStr=boolean
  Sum : Sum  Inputs=|+-  OutDataTypeStr=int32
  Sum1 : Sum  Inputs=|++
  Switch : Switch  Criteria=u2 > Threshold  Threshold=eps  SaturateOnIntegerOverflow=off  InputSameDT=off
  Unit Delay : UnitDelay  SampleTime=dt0  HasFrameUpgradeWarning=on
  Unit Delay1 : UnitDelay  SampleTime=dt0  HasFrameUpgradeWarning=on
  Unit Delay2 : UnitDelay  SampleTime=dt0  HasFrameUpgradeWarning=on
  Out1 : Outport
  wires:
  Logical Operator/1 -> Unit Delay2/1, Out1/1
  Constant1/1 -> Sum1/1
  Compare To Constant/1 -> Logical Operator/1
  Switch/1 -> Unit Delay1/1, Compare To Constant/1
  In1/1 -> Sum/1, Unit Delay/1
  Unit Delay2/1 -> Logical Operator/2
  Unit Delay/1 -> Sum/2
  Sum/1 -> Switch/2
  Sum1/1 -> Switch/3
  Unit Delay1/1 -> Sum1/2
  Constant/1 -> Switch/1

== system Bossi_Emanuele_EE460S3D_R99/S3D_Plant/Sensors/HealthMonitoring/Subsystem5 ==
  In1 : Inport
  Compare To Constant : simulink/Logic and Bit Operations/Compare To Constant  relop=>=  const=HM_S  OutDataTypeStr=boolean
  Constant : Constant  Value=0
  Constant1 : Constant
  Logical Operator : Logic  Operator=OR  AllPortsSameDT=off  OutDataTypeStr=boolean
  Sum : Sum  Inputs=|+-  OutDataTypeStr=int32
  Sum1 : Sum  Inputs=|++
  Switch : Switch  Criteria=u2 > Threshold  Threshold=eps  SaturateOnIntegerOverflow=off  InputSameDT=off
  Unit Delay : UnitDelay  SampleTime=dt0  HasFrameUpgradeWarning=on
  Unit Delay1 : UnitDelay  SampleTime=dt0  HasFrameUpgradeWarning=on
  Unit Delay2 : UnitDelay  SampleTime=dt0  HasFrameUpgradeWarning=on
  Out1 : Outport
  wires:
  Constant/1 -> Switch/1
  Unit Delay1/1 -> Sum1/2
  Sum1/1 -> Switch/3
  Sum/1 -> Switch/2
  Unit Delay/1 -> Sum/2
  Unit Delay2/1 -> Logical Operator/2
  In1/1 -> Unit Delay/1, Sum/1
  Switch/1 -> Compare To Constant/1, Unit Delay1/1
  Compare To Constant/1 -> Logical Operator/1
  Constant1/1 -> Sum1/1
  Logical Operator/1 -> Out1/1, Unit Delay2/1

== system Bossi_Emanuele_EE460S3D_R99/S3D_Plant/Sensors/HealthMonitoring/Subsystem6 ==
  In1 : Inport
  Compare To Constant : simulink/Logic and Bit Operations/Compare To Constant  relop=>=  const=HM_S  OutDataTypeStr=boolean
  Constant : Constant  Value=0
  Constant1 : Constant
  Logical Operator : Logic  Operator=OR  AllPortsSameDT=off  OutDataTypeStr=boolean
  Sum : Sum  Inputs=|+-  OutDataTypeStr=int32
  Sum1 : Sum  Inputs=|++
  Switch : Switch  Criteria=u2 > Threshold  Threshold=eps  SaturateOnIntegerOverflow=off  InputSameDT=off
  Unit Delay : UnitDelay  SampleTime=dt0  HasFrameUpgradeWarning=on
  Unit Delay1 : UnitDelay  SampleTime=dt0  HasFrameUpgradeWarning=on
  Unit Delay2 : UnitDelay  SampleTime=dt0  HasFrameUpgradeWarning=on
  Out1 : Outport
  wires:
  Logical Operator/1 -> Unit Delay2/1, Out1/1
  Constant1/1 -> Sum1/1
  Compare To Constant/1 -> Logical Operator/1
  Switch/1 -> Unit Delay1/1, Compare To Constant/1
  In1/1 -> Sum/1, Unit Delay/1
  Unit Delay2/1 -> Logical Operator/2
  Unit Delay/1 -> Sum/2
  Sum/1 -> Switch/2
  Sum1/1 -> Switch/3
  Unit Delay1/1 -> Sum1/2
  Constant/1 -> Switch/1

== system Bossi_Emanuele_EE460S3D_R99/S3D_Plant/Sensors/HealthMonitoring/Subsystem7 ==
  In1 : Inport
  Compare To Constant : simulink/Logic and Bit Operations/Compare To Constant  relop=>=  const=HM_S  OutDataTypeStr=boolean
  Constant : Constant  Value=0
  Constant1 : Constant
  Logical Operator : Logic  Operator=OR  AllPortsSameDT=off  OutDataTypeStr=boolean
  Sum : Sum  Inputs=|+-  OutDataTypeStr=int32
  Sum1 : Sum  Inputs=|++
  Switch : Switch  Criteria=u2 > Threshold  Threshold=eps  SaturateOnIntegerOverflow=off  InputSameDT=off
  Unit Delay : UnitDelay  SampleTime=dt0  HasFrameUpgradeWarning=on
  Unit Delay1 : UnitDelay  SampleTime=dt0  HasFrameUpgradeWarning=on
  Unit Delay2 : UnitDelay  SampleTime=dt0  HasFrameUpgradeWarning=on
  Out1 : Outport
  wires:
  Constant/1 -> Switch/1
  Unit Delay1/1 -> Sum1/2
  Sum1/1 -> Switch/3
  Sum/1 -> Switch/2
  Unit Delay/1 -> Sum/2
  Unit Delay2/1 -> Logical Operator/2
  In1/1 -> Unit Delay/1, Sum/1
  Switch/1 -> Compare To Constant/1, Unit Delay1/1
  Compare To Constant/1 -> Logical Operator/1
  Constant1/1 -> Sum1/1
  Logical Operator/1 -> Out1/1, Unit Delay2/1

== system Bossi_Emanuele_EE460S3D_R99/S3D_Plant/Sensors/HealthMonitoring/Subsystem8 ==
  In1 : Inport
  Compare To Constant : simulink/Logic and Bit Operations/Compare To Constant  relop=>=  const=HM_S  OutDataTypeStr=boolean
  Constant : Constant  Value=0
  Constant1 : Constant
  Logical Operator : Logic  Operator=OR  AllPortsSameDT=off  OutDataTypeStr=boolean
  Sum : Sum  Inputs=|+-  OutDataTypeStr=int32
  Sum1 : Sum  Inputs=|++
  Switch : Switch  Criteria=u2 > Threshold  Threshold=eps  SaturateOnIntegerOverflow=off  InputSameDT=off
  Unit Delay : UnitDelay  SampleTime=dt0  HasFrameUpgradeWarning=on
  Unit Delay1 : UnitDelay  SampleTime=dt0  HasFrameUpgradeWarning=on
  Unit Delay2 : UnitDelay  SampleTime=dt0  HasFrameUpgradeWarning=on
  Out1 : Outport
  wires:
  Logical Operator/1 -> Unit Delay2/1, Out1/1
  Constant1/1 -> Sum1/1
  Compare To Constant/1 -> Logical Operator/1
  Switch/1 -> Unit Delay1/1, Compare To Constant/1
  In1/1 -> Sum/1, Unit Delay/1
  Unit Delay2/1 -> Logical Operator/2
  Unit Delay/1 -> Sum/2
  Sum/1 -> Switch/2
  Sum1/1 -> Switch/3
  Unit Delay1/1 -> Sum1/2
  Constant/1 -> Switch/1

== system Bossi_Emanuele_EE460S3D_R99/S3D_Plant/ThrusterValues/FailModes/Ufail1 ==
  Uin : Inport
  MP : Inport  Port=2
  Bus Selector1 : BusSelector  OutputSignals=U1cmd,U2cmd,U3cmd,U4cmd,U5cmd,U6cmd,U7cmd,U8cmd,U9cmd,U10cmd  OutputAsBus=on
  Bus Selector2 : BusSelector  OutputSignals=MfuelVector
  Bus to Vector2 : BusToVector
  CURRENT : Subsystem  TreatAsAtomicUnit=on
  Compare To Constant2 : simulink/Logic and Bit Operations/Compare To Constant  relop=>  const=eps  OutDataTypeStr=boolean
  Constant2 : Constant  Value=LVL.Uft(Udx,1)+rand*(LVL.Uft(Udx,2)-LVL.Uft(Udx,1))  SampleTime=dt0
  Constant3 : Constant  Value=LVL.Ufail(Udx)  SampleTime=dt0
  Constant4 : Constant  Value=-1  SampleTime=dt0
  Digital Clock : DigitalClock  SampleTime=dt0
  FailLogic : Subsystem
  If : If  IfExpression=u1 < -0.5  ElseIfExpressions=u1 > 0.5 & u1 < 1.5  SampleTime=dt0
  MAX : Subsystem  TreatAsAtomicUnit=on
  MIN : Subsystem  TreatAsAtomicUnit=on
  Merge : Merge  Inputs=3
  Relational Operator : RelationalOperator  Operator=<  OutDataTypeStr=boolean  InputSameDT=off
  Selector1 : Selector  InputPortWidth=4  IndexOptions=Index vector (dialog)  Indices=[Tank]  OutputSizes=1
  Selector2 : Selector  InputPortWidth=10  IndexOptions=Index vector (dialog)  Indices=[Udx]  OutputSizes=1
  Switch : Switch  Criteria=u2 > Threshold  SaturateOnIntegerOverflow=off  InputSameDT=off
  Switch1 : Switch  Criteria=u2 > Threshold  SaturateOnIntegerOverflow=off  InputSameDT=off
  Unit Delay : UnitDelay  SampleTime=dt0  HasFrameUpgradeWarning=on
  Uout : Outport
  wires:
  Selector2/1 -> Switch/1
  Bus to Vector2/1 -> Selector2/1
  FailLogic/1(NoFail) -> Switch/2
  Compare To Constant2/1 -> Switch1/2, FailLogic/2(FuelRemaining)
  Relational Operator/1 -> FailLogic/1(BeforeFail)
  Constant4/1 -> Switch1/3
  Constant3/1 -> Switch1/1
  Selector1/1 -> Compare To Constant2/1
  Bus Selector2/1 -> Selector1/1  "<MfuelVector>"
  MP/1 -> Bus Selector2/1
  Bus Selector1/1 -> Bus to Vector2/1
  Switch/1 -> Unit Delay/1, Uout/1
  Switch1/1 -> If/1, FailLogic/3(FailMode)
  Uin/1 -> Bus Selector1/1
  Merge/1 -> Switch/3
  MIN/1(Out1) -> Merge/1
  CURRENT/1(Out1) -> Merge/3
  Constant2/1 -> Relational Operator/2
  MAX/1(Out1) -> Merge/2
  Unit Delay/1 -> CURRENT/1(In1)
  If/3 -> CURRENT/Action
  Digital Clock/1 -> Relational Operator/1
  If/2 -> MAX/Action
  If/1 -> MIN/Action

== system Bossi_Emanuele_EE460S3D_R99/S3D_Plant/ThrusterValues/FailModes/Ufail10 ==
  Uin : Inport
  Bus Selector1 : BusSelector  OutputSignals=U1cmd,U2cmd,U3cmd,U4cmd,U5cmd,U6cmd,U7cmd,U8cmd,U9cmd,U10cmd  OutputAsBus=on
  Bus to Vector2 : BusToVector
  CURRENT : Subsystem  TreatAsAtomicUnit=on
  Constant1 : Constant  OutDataTypeStr=boolean  SampleTime=dt0
  Constant2 : Constant  Value=LVL.Uft(Udx,1)+rand*(LVL.Uft(Udx,2)-LVL.Uft(Udx,1))  SampleTime=dt0
  Constant3 : Constant  Value=LVL.Ufail(Udx)  SampleTime=dt0
  Constant4 : Constant  Value=-1  SampleTime=dt0
  Digital Clock : DigitalClock  SampleTime=dt0
  FailLogic : Subsystem
  If : If  IfExpression=u1 < -0.5  ElseIfExpressions=u1 > 0.5 & u1 < 1.5  SampleTime=dt0
  MAX : Subsystem  TreatAsAtomicUnit=on
  MIN : Subsystem  TreatAsAtomicUnit=on
  Merge : Merge  Inputs=3
  Relational Operator : RelationalOperator  Operator=<  OutDataTypeStr=boolean  InputSameDT=off
  Selector2 : Selector  InputPortWidth=10  IndexOptions=Index vector (dialog)  Indices=[Udx]  OutputSizes=1
  Switch : Switch  Criteria=u2 > Threshold  SaturateOnIntegerOverflow=off  InputSameDT=off
  Switch1 : Switch  Criteria=u2 > Threshold  SaturateOnIntegerOverflow=off  InputSameDT=off
  Unit Delay : UnitDelay  SampleTime=dt0  HasFrameUpgradeWarning=on
  Uout : Outport
  wires:
  Selector2/1 -> Switch/1
  Bus to Vector2/1 -> Selector2/1
  Bus Selector1/1 -> Bus to Vector2/1
  FailLogic/1(NoFail) -> Switch/2
  Constant1/1 -> Switch1/2, FailLogic/2(FuelRemaining)
  Relational Operator/1 -> FailLogic/1(BeforeFail)
  Constant4/1 -> Switch1/3
  Constant3/1 -> Switch1/1
  Switch/1 -> Unit Delay/1, Uout/1
  Switch1/1 -> If/1, FailLogic/3(FailMode)
  Uin/1 -> Bus Selector1/1
  Merge/1 -> Switch/3
  MIN/1(Out1) -> Merge/1
  CURRENT/1(Out1) -> Merge/3
  Constant2/1 -> Relational Operator/2
  MAX/1(Out1) -> Merge/2
  Unit Delay/1 -> CURRENT/1(In1)
  If/3 -> CURRENT/Action
  Digital Clock/1 -> Relational Operator/1
  If/2 -> MAX/Action
  If/1 -> MIN/Action

== system Bossi_Emanuele_EE460S3D_R99/S3D_Plant/ThrusterValues/FailModes/Ufail2 ==
  Uin : Inport
  MP : Inport  Port=2
  Bus Selector1 : BusSelector  OutputSignals=U1cmd,U2cmd,U3cmd,U4cmd,U5cmd,U6cmd,U7cmd,U8cmd,U9cmd,U10cmd  OutputAsBus=on
  Bus Selector2 : BusSelector  OutputSignals=MfuelVector
  Bus to Vector2 : BusToVector
  CURRENT : Subsystem  TreatAsAtomicUnit=on
  Compare To Constant2 : simulink/Logic and Bit Operations/Compare To Constant  relop=>  const=eps  OutDataTypeStr=boolean
  Constant2 : Constant  Value=LVL.Uft(Udx,1)+rand*(LVL.Uft(Udx,2)-LVL.Uft(Udx,1))  SampleTime=dt0
  Constant3 : Constant  Value=LVL.Ufail(Udx)  SampleTime=dt0
  Constant4 : Constant  Value=-1  SampleTime=dt0
  Digital Clock : DigitalClock  SampleTime=dt0
  FailLogic : Subsystem
  If : If  IfExpression=u1 < -0.5  ElseIfExpressions=u1 > 0.5 & u1 < 1.5  SampleTime=dt0
  MAX : Subsystem  TreatAsAtomicUnit=on
  MIN : Subsystem  TreatAsAtomicUnit=on
  Merge : Merge  Inputs=3
  Relational Operator : RelationalOperator  Operator=<  OutDataTypeStr=boolean  InputSameDT=off
  Selector1 : Selector  InputPortWidth=4  IndexOptions=Index vector (dialog)  Indices=[Tank]  OutputSizes=1
  Selector2 : Selector  InputPortWidth=10  IndexOptions=Index vector (dialog)  Indices=[Udx]  OutputSizes=1
  Switch : Switch  Criteria=u2 > Threshold  SaturateOnIntegerOverflow=off  InputSameDT=off
  Switch1 : Switch  Criteria=u2 > Threshold  SaturateOnIntegerOverflow=off  InputSameDT=off
  Unit Delay : UnitDelay  SampleTime=dt0  HasFrameUpgradeWarning=on
  Uout : Outport
  wires:
  Selector2/1 -> Switch/1
  Bus to Vector2/1 -> Selector2/1
  Bus Selector1/1 -> Bus to Vector2/1
  FailLogic/1(NoFail) -> Switch/2
  Compare To Constant2/1 -> Switch1/2, FailLogic/2(FuelRemaining)
  Relational Operator/1 -> FailLogic/1(BeforeFail)
  Constant4/1 -> Switch1/3
  Constant3/1 -> Switch1/1
  Selector1/1 -> Compare To Constant2/1
  Bus Selector2/1 -> Selector1/1  "<MfuelVector>"
  MP/1 -> Bus Selector2/1
  Switch/1 -> Unit Delay/1, Uout/1
  Switch1/1 -> If/1, FailLogic/3(FailMode)
  Uin/1 -> Bus Selector1/1
  Merge/1 -> Switch/3
  MIN/1(Out1) -> Merge/1
  CURRENT/1(Out1) -> Merge/3
  Constant2/1 -> Relational Operator/2
  MAX/1(Out1) -> Merge/2
  Unit Delay/1 -> CURRENT/1(In1)
  If/3 -> CURRENT/Action
  Digital Clock/1 -> Relational Operator/1
  If/2 -> MAX/Action
  If/1 -> MIN/Action

== system Bossi_Emanuele_EE460S3D_R99/S3D_Plant/ThrusterValues/FailModes/Ufail3 ==
  Uin : Inport
  MP : Inport  Port=2
  Bus Selector1 : BusSelector  OutputSignals=U1cmd,U2cmd,U3cmd,U4cmd,U5cmd,U6cmd,U7cmd,U8cmd,U9cmd,U10cmd  OutputAsBus=on
  Bus Selector2 : BusSelector  OutputSignals=MfuelVector
  Bus to Vector2 : BusToVector
  CURRENT : Subsystem  TreatAsAtomicUnit=on
  Compare To Constant2 : simulink/Logic and Bit Operations/Compare To Constant  relop=>  const=eps  OutDataTypeStr=boolean
  Constant2 : Constant  Value=LVL.Uft(Udx,1)+rand*(LVL.Uft(Udx,2)-LVL.Uft(Udx,1))  SampleTime=dt0
  Constant3 : Constant  Value=LVL.Ufail(Udx)  SampleTime=dt0
  Constant4 : Constant  Value=-1  SampleTime=dt0
  Digital Clock : DigitalClock  SampleTime=dt0
  FailLogic : Subsystem
  If : If  IfExpression=u1 < -0.5  ElseIfExpressions=u1 > 0.5 & u1 < 1.5  SampleTime=dt0
  MAX : Subsystem  TreatAsAtomicUnit=on
  MIN : Subsystem  TreatAsAtomicUnit=on
  Merge : Merge  Inputs=3
  Relational Operator : RelationalOperator  Operator=<  OutDataTypeStr=boolean  InputSameDT=off
  Selector1 : Selector  InputPortWidth=4  IndexOptions=Index vector (dialog)  Indices=[Tank]  OutputSizes=1
  Selector2 : Selector  InputPortWidth=10  IndexOptions=Index vector (dialog)  Indices=[Udx]  OutputSizes=1
  Switch : Switch  Criteria=u2 > Threshold  SaturateOnIntegerOverflow=off  InputSameDT=off
  Switch1 : Switch  Criteria=u2 > Threshold  SaturateOnIntegerOverflow=off  InputSameDT=off
  Unit Delay : UnitDelay  SampleTime=dt0  HasFrameUpgradeWarning=on
  Uout : Outport
  wires:
  Selector2/1 -> Switch/1
  Bus to Vector2/1 -> Selector2/1
  Bus Selector1/1 -> Bus to Vector2/1
  FailLogic/1(NoFail) -> Switch/2
  Compare To Constant2/1 -> Switch1/2, FailLogic/2(FuelRemaining)
  Relational Operator/1 -> FailLogic/1(BeforeFail)
  Constant4/1 -> Switch1/3
  Constant3/1 -> Switch1/1
  Selector1/1 -> Compare To Constant2/1
  Bus Selector2/1 -> Selector1/1  "<MfuelVector>"
  MP/1 -> Bus Selector2/1
  Switch/1 -> Unit Delay/1, Uout/1
  Switch1/1 -> If/1, FailLogic/3(FailMode)
  Uin/1 -> Bus Selector1/1
  Merge/1 -> Switch/3
  MIN/1(Out1) -> Merge/1
  CURRENT/1(Out1) -> Merge/3
  Constant2/1 -> Relational Operator/2
  MAX/1(Out1) -> Merge/2
  Unit Delay/1 -> CURRENT/1(In1)
  If/3 -> CURRENT/Action
  Digital Clock/1 -> Relational Operator/1
  If/2 -> MAX/Action
  If/1 -> MIN/Action
